simulink model "sschdlexSolarInverterSingleNetworkModel"  (R2026a)
settings: Solver=FixedStepDiscrete  StopTime=.5  MaxStep=1e-4
PreLoadFcn:
  | load('EmulatedPV_LowPowerData.mat');
  | irr = 0.15;
  | numIrr = 10;
  | ArrayPower = ArrayCurrent.*ArrayVoltage;
  | 
  | C_Boost_In = 680e-6;
  | C_Boost_In_R = 0;
  | L_Boost = 100e-6;
  | L_Boost_R = 0;
  | C_Boost_Out = 1640e-6;
  | 
  | TsFPGA = 2e-6;
  | TsControl = 2e-6;
  | TsCPU = 2e-6;
  | Tc = TsControl;
  | Ts = 2e-6;
  | 
  | IGBT_Vth = 6;
  | IGBT_Vf = 0.8;
  | IGBT_R = 0.001;
  | IGBT_Con = 1e-5;
  | 
  | IGBT_D_Vth = 0.8;
  | IGBT_D_R = 0.001;
  | IGBT_D_Con = 1e-5;
  | 
  | maxIn = 10;
  | minIn = -10;
  | maxOut = 2^15;
  | minOut = -2^15;
  | difIn = maxIn-minIn;
  | difOut = maxOut-minOut;
  | gain = difOut/difIn;
  | dc1 = (maxOut+minOut)/2;
  | dc2 = (maxIn+minIn)/2;
  | offset = dc1-gain*dc2;
  | numIrr = 10;
  | ArrayPower = ArrayCurrent.*ArrayVoltage;
InitFcn:
  | Ts = 2e-6;
  | Tc = Ts;
values from neighbouring files (symbols this model uses):
  ArrayCurrent = [3 2.90135967378 2.78442846347 2.64406556825 2.47269969012 2.25842875672 1.98100825201 1.60223040661 1.04533074246 0.222841716608 0 0 ... (1000 elements, 100x10)]    [EmulatedPV_LowPowerData.mat]
  ArrayVoltage = [0 0.151515151515 0.30303030303 0.454545454545 0.606060606061 0.757575757576 0.909090909091 1.06060606061 1.21212121212 1.36363636364 1.51515151515 1.66666666667 ... (100 elements, 100x1)]    [EmulatedPV_LowPowerData.mat]
  Irradiance = [0.05 0.1 0.15 0.2 0.25 0.3 0.35 0.4 0.45 0.5]    [EmulatedPV_LowPowerData.mat]
undefined symbols (not defined in the file or in its folder): DiscIntNeverNeededParam, ee_sli_rtmsupport, gcbh, Tdata
libraries: fl_lib x19, nesl_utility x12, eeGeneralControl x8, ee_lib x6, simulink x3, slpidlib x2
(part 1 of 2)
CloseFcn:
  | clear ArrayCurrent
  | clear ArrayVoltage
  | clear Irradiance
  | 
  | clear irr;
  | clear numIrr;
  | clear ArrayPower;
  | 
  | clear C_Boost_In;
  | clear C_Boost_In_R;
  | clear L_Boost;
  | clear L_Boost_R;
  | clear C_Boost_Out;
  | 
  | clear TsFPGA;
  | clear TsControl;
  | clear TsCPU;
  | clear Tc;
  | clear Ts;
  | 
  | clear IGBT_Vth;
  | clear IGBT_Vf;
  | clear IGBT_R ;
  | clear IGBT_Con;
  | 
  | clear IGBT_D_Vth;
  | clear IGBT_D_R;
  | clear IGBT_D_Con;
  | 
  | clear maxIn;
  | clear minIn;
  | clear maxOut;
  | clear minOut;
  | clear difIn;
  | clear difOut;
  | clear gain;
  | clear dc1;
  | clear dc2;
  | clear offset;
settings Model: DataTypeOverride=Off  Creator=The MathWorks, Inc.  LastModifiedBy=The MathWorks, Inc.
settings OptimizationCC: ConditionallyExecuteInputs=off  InheritOutputTypeSmallerThanSingle=on  EfficientMapNaN2IntZero=off
settings DebuggingCC: ArtificialAlgebraicLoopMsg=error  SingleTaskRateTransMsg=error  ParameterPrecisionLossMsg=none  PregeneratedLibrarySubsystemCodeDiagnostic=none
settings HardwareCC: ProdHWDeviceType=ASIC/FPGA->ASIC/FPGA  TargetBitPerLong=64.0  TargetBitPerPointer=64.0  TargetBitPerSizeT=64.0  TargetBitPerPtrDiffT=64.0  TargetLongLongMode=on  TargetIntDivRoundTo=Zero  TargetEndianess=LittleEndian  TargetWordSize=64.0  TargetHWDeviceType=Custom Processor->MATLAB Host Computer  ProdEqTarget=off
settings CodeAppCC: MaxIdLength=128.0
settings GRTTargetCC: CombineOutputUpdateFcns=off  GRTInterface=on
settings SimscapeCC: SimscapeNominalValues="[{\"value\":\"1\",\"unit\":\"A\"},{\"value\":\"1\",\"unit\":\"bar\"},{\"value\":\"1\",\"unit\":\"cm^2\"},{\"value\":\"1\",\"unit\":\"cm^3/s\"},{\"value\":\"1\",\"unit\":\"kJ/kg\"},{\"value\":\"1\",\"unit\":\"kW\"},{\"value\":\"1\",\"unit\":\"l\"},{\"value\":\"1\",\"unit\":\"N\"},{\"value\":\"1\",\"unit\":\"N*m\"},{\"value\":\"1\",\"unit\":\"V\"}]"  SimscapeLogType=none  SimscapeLogDataHistory=5000.0

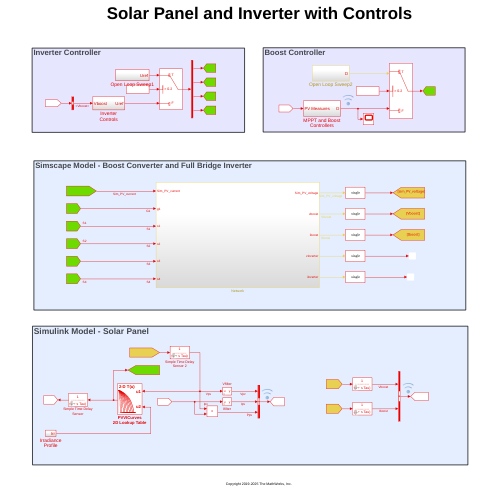
[thumbnail: Simulink's stored preview of the top-level diagram]
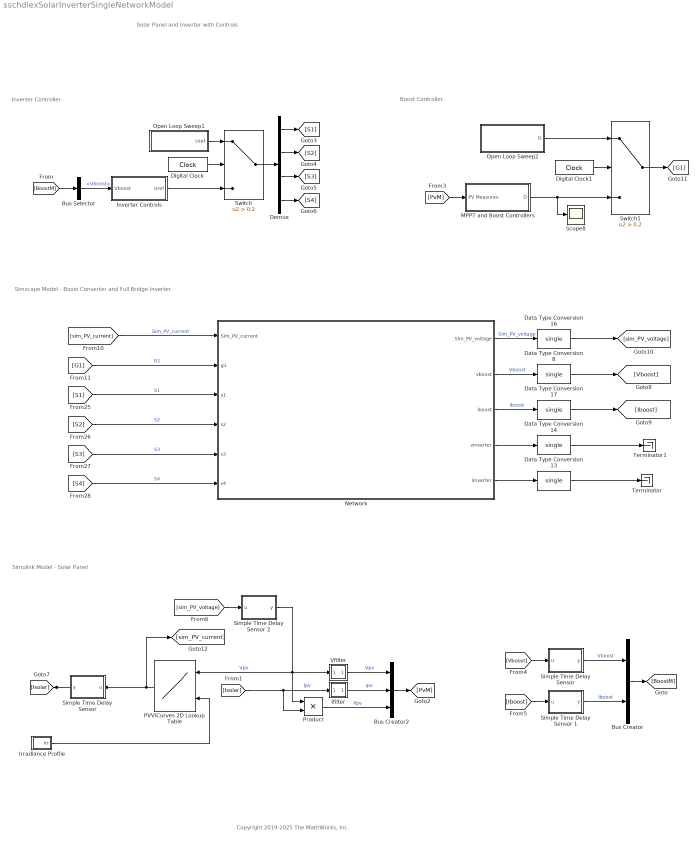
== system sschdlexSolarInverterSingleNetworkModel ==
  note: Solar Panel and Inverter with Controls
  note: Simulink Model - Solar Panel
  note: Inverter Controller
  note: Boost Controller
  note: Simscape Model - Boost Converter and Full Bridge Inverter
  note: Copyright 2019-2025 The MathWorks, Inc.
  Bus Creator : BusCreator  Inputs=2
  Bus Creator2 : BusCreator  Inputs=3
  Bus Selector : BusSelector  OutputSignals=Vboost
  Data Type Conversion{13..14,16..17} (4 alike) : DataTypeConversion  OutDataTypeStr=single  RndMeth=Nearest  SaturateOnIntegerOverflow=off
  Data Type Conversion8 : DataTypeConversion  OutDataTypeStr=single  SaturateOnIntegerOverflow=off  RndMeth=Floor
  Demux : Demux
  Digital Clock : DigitalClock  SampleTime=2e-6
  Digital Clock1 : DigitalClock  SampleTime=2e-6
  Ifilter : Subsystem  mask{Tf=0.01}
      mask prompts: Tf "Filter Time Constant"
  Inverter Controls : Subsystem
  Irradiance Profile : Subsystem
  MPPT and Boost Controllers : Subsystem
  Network : Subsystem
  Open Loop Sweep1 : Subsystem
  Open Loop Sweep2 : Subsystem
  PVVICurves 2D Lookup Table : Lookup_n-D  BreakpointsForDimension1=ArrayVoltage  BreakpointsForDimension2=Irradiance  Table=ArrayCurrent  InternalRulePriority=Speed  RndMeth=Simplest
      settings: InputPortMap=u0,u1
  Product : Product
  Scope8 : Scope
  Simple Time Delay Sensor : Subsystem  mask{Ts=Ts, Tau=0.0001}
      mask prompts: Ts "Sample Time, [s]"; Tau "Time Constant, Tau [s]"
      mask help: Simple Sensor
      mask Display: fprintf('1\n------------\n(1 + s Tau)');
  "Simple Time Delay Sensor " : Subsystem  mask{Ts=Ts, Tau=0.0001}
      mask prompts: Ts "Sample Time, [s]"; Tau "Time Constant, Tau [s]"
      mask help: Simple Sensor
      mask Display: fprintf('1\n------------\n(1 + s Tau)');
  Simple Time Delay Sensor 1 : Subsystem  mask{Ts=Ts, Tau=0.0001}
      mask prompts: Ts "Sample Time, [s]"; Tau "Time Constant, Tau [s]"
      mask help: Simple Sensor
      mask Display: fprintf('1\n------------\n(1 + s Tau)');
  Simple Time Delay Sensor 2 : Subsystem  mask{Ts=Ts, Tau=0.0001}
      mask prompts: Ts "Sample Time, [s]"; Tau "Time Constant, Tau [s]"
      mask help: Simple Sensor
      mask Display: fprintf('1\n------------\n(1 + s Tau)');
  Switch : Switch  Criteria=u2 > Threshold  Threshold=0.2  SaturateOnIntegerOverflow=off  InputSameDT=off
  Switch1 : Switch  Criteria=u2 > Threshold  Threshold=0.2  SaturateOnIntegerOverflow=off  InputSameDT=off
  Terminator : Terminator
  Terminator1 : Terminator
  Vfilter : Subsystem  mask{Tf=0.01}
      mask prompts: Tf "Filter Time Constant"
  wires:
  Bus Creator/1 -> [BoostM]
  Demux/3 -> [S3]
  Demux/2 -> [S2]
  Irradiance Profile/1(Irr) -> PVVICurves 2D Lookup Table/2
  Product/1 -> Bus Creator2/3  "Ppv"
  Vfilter/1(y) -> Bus Creator2/1  "Vpv"
  [PvM] -> MPPT and Boost Controllers/1(PV Measures)
  PVVICurves 2D Lookup Table/1 -> Simple Time Delay Sensor/1(u), [sim_PV_current]
  [sim_PV_voltage] -> Simple Time Delay Sensor 2/1(u)
  MPPT and Boost Controllers/1(D) -> Scope8/1, Switch1/3
  [Iboost] -> Simple Time Delay Sensor 1/1(u)
  Open Loop Sweep1/1(Uref) -> Switch/1
  Bus Selector/1 -> Inverter Controls/1(Vboost)  "<Vboost>"
  Digital Clock1/1 -> Switch1/2
  Ifilter/1(y) -> Bus Creator2/2  "Ipv"
  [Isolar] -> Product/2, Ifilter/1(u)  "Ipv"
  Switch/1 -> Demux/1
  Switch1/1 -> [G1]
  Simple Time Delay Sensor/1(y) -> [Isolar]
  Bus Creator2/1 -> [PvM]
  Simple Time Delay Sensor 2/1(y) -> PVVICurves 2D Lookup Table/1, Product/1, Vfilter/1(u)  "Vpv"
  Simple Time Delay Sensor 1/1(y) -> Bus Creator/2  "Iboost"
  [Vboost] -> "Simple Time Delay Sensor "/1(u)
  Demux/1 -> [S1]
  Demux/4 -> [S4]
  [BoostM] -> Bus Selector/1
  Open Loop Sweep2/1(D) -> Switch1/1
  "Simple Time Delay Sensor "/1(y) -> Bus Creator/1  "Vboost"
  Inverter Controls/1(Uref) -> Switch/3
  Digital Clock/1 -> Switch/2
  [S4] -> Network/6(s4)  "S4"
  [S2] -> Network/4(s2)  "S2"
  [S1] -> Network/3(s1)  "S1"
  Data Type Conversion8/1 -> [Vboost]
  Data Type Conversion16/1 -> [sim_PV_voltage]
  Data Type Conversion17/1 -> [Iboost]
  [sim_PV_current] -> Network/1(Sim_PV_current)  "Sim_PV_current"
  Network/1(Sim_PV_voltage) -> Data Type Conversion16/1  "Sim_PV_voltage"
  Network/3(iboost) -> Data Type Conversion17/1  "Iboost"
  Network/2(vboost) -> Data Type Conversion8/1  "Vboost"
  [G1] -> Network/2(g1)  "G1"
  Data Type Conversion13/1 -> Terminator/1
  Data Type Conversion14/1 -> Terminator1/1
  [S3] -> Network/5(s3)  "S3"
  Network/4(vinverter) -> Data Type Conversion14/1
  Network/5(iinverter) -> Data Type Conversion13/1

== system sschdlexSolarInverterSingleNetworkModel/Ifilter ==
  u : Inport
  1/T6 : Gain  Gain=1/Tf
  Discrete-Time Integrator : DiscreteIntegrator  SampleTime=Tc  ICPrevOutput=DiscIntNeverNeededParam  ICPrevScaledInput=DiscIntNeverNeededParam
  Sum1 : Sum  Inputs=|+-
  y : Outport  VectorParamsAs1DForOutWhenUnconnected=off
  wires:
  Sum1/1 -> 1/T6/1
  Discrete-Time Integrator/1 -> Sum1/2, y/1
  u/1 -> Sum1/1
  1/T6/1 -> Discrete-Time Integrator/1

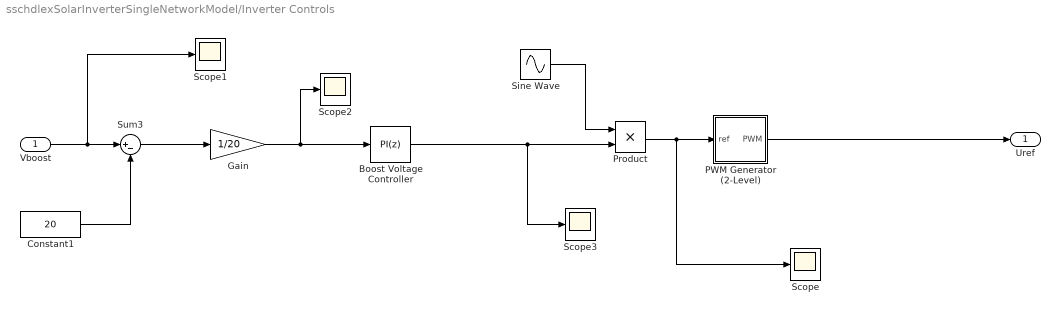
== system sschdlexSolarInverterSingleNetworkModel/Inverter Controls ==
  Vboost : Inport
  Boost Voltage Controller : slpidlib/PID Controller  Controller=PI  Form=Parallel  TimeDomain=Discrete-time  UseExternalTs=off  SampleTime=Tc  IntegratorMethod=Forward Euler  FilterMethod=Forward Euler  ControllerParametersSource=internal  P=4  I=500  UseKiTs=off  D=0  UseExternalDerivativeSource=off  N=100  UseFilter=on  TunerSelectOption=Transfer Function Based (PID Tuner App)  InitialConditionSource=internal  InitialConditionForIntegrator=1  InitialConditionForFilter=0  DifferentiatorICPrevScaledInput=0  ExternalReset=none  TrackingMode=off  Kt=1  LimitOutput=on  SatLimitsSource=internal  UpperSaturationLimit=1  LowerSaturationLimit=0  LinearizeAsGain=on  AntiWindupMode=clamping  Kb=1  LimitIntegrator=off  UpperIntegratorSaturationLimit=inf  LowerIntegratorSaturationLimit=-inf  POutMin=[]  POutMax=[]  IOutMin=[]  IOutMax=[]  DOutMin=[]  DOutMax=[]  NOutMin=[]  NOutMax=[]  SumOutMin=[]  SumOutMax=[]  SaturationOutMin=[]  SaturationOutMax=[]  PParamMin=[]  PParamMax=[]  IParamMin=[]  IParamMax=[]  DParamMin=[]  DParamMax=[]  NParamMin=[]  NParamMax=[]  KbParamMin=[]  KbParamMax=[]  KtParamMin=[]  KtParamMax=[]  KbOutMin=[]  KbOutMax=[]  KtOutMin=[]  KtOutMax=[]  IntegratorOutMin=[]  IntegratorOutMax=[]  FilterOutMin=[]  FilterOutMax=[]  SumI1OutMin=[]  SumI1OutMax=[]  SumI2OutMin=[]  SumI2OutMax=[]  SumI3OutMin=[]  SumI3OutMax=[]  SumI4OutMin=[]  SumI4OutMax=[]  SumDOutMin=[]  SumDOutMax=[]  DifferentiatorOutMin=[]  DifferentiatorOutMax=[]  FilterDiffOutCoefMin=[]  FilterDiffOutCoefMax=[]  ReciprocalOutMin=[]  ReciprocalOutMax=[]  SumDenOutMin=[]  SumDenOutMax=[]  SumNumOutMin=[]  SumNumOutMax=[]  DivideOutMin=[]  DivideOutMax=[]  UdiffTsProdOutMin=[]  UdiffTsProdOutMax=[]  NTsProdOutMin=[]  NTsProdOutMax=[]  UintegralTsProdOutMin=[]  UintegralTsProdOutMax=[]  UngainTsProdOutMin=[]  UngainTsProdOutMax=[]  ClampingZeroOutDataTypeStr=Inherit: Inherit via back propagation  ClampingZeroOutMin=[]  ClampingZeroOutMax=[]  FilterDenConstantOutDataTypeStr=Inherit: Inherit via back propagation  FilterDenConstantOutMin=[]  FilterDenConstantOutMax=[]  PCopyOutDataTypeStr=Inherit: Inherit via back propagation  PCopyOutMin=[]  PCopyOutMax=[]  NCopyOutDataTypeStr=Inherit: Inherit via back propagation  NCopyOutMin=[]  NCopyOutMax=[]  IntegratorContinuousStateAttributes=''  IntegratorStateMustResolveToSignalObject=off  IntegratorRTWStateStorageClass=Auto  FilterContinuousStateAttributes=''  FilterStateMustResolveToSignalObject=off  FilterRTWStateStorageClass=Auto  ParallelPVariant=InternalParameters  IdealPVariant=Disabled  IVariant=InternalParameters  DVariant=Disabled  IntegratorVariant=Discrete  SatVariant=Enabled  AWVariant=DiscClampingParallel  PCopyVariant=Disabled  TRVariant=Disabled  FdbkBlocksVariant=Forward  IdealPFdbkVariant=Disabled  SatFdbkVariant=Disabled  DerivativeFilterVariant=Disabled  NVariant=Disabled  NCopyVariant=Disabled_SignalSpec  FilterICVariant=Disabled  IntegratorICVariant=InternalICs  ExternalResetVariant=Disabled  TRSumVariant=Passthrough  SumFdbkVariant=Disabled  SumVariant=Sum_PI  TsampFilterVariant=InternalTs  TsampNgainVariant=Passthrough  TsampIntegralVariant=Disabled_SignalSpec  ExternalSaturationOutDataTypeStr=Inherit: Same as second input  DerivativeSourceVariant=Disabled  PreIntVariant=InternalPreInt
  Constant1 : Constant  Value=20
  Gain : Gain  Gain=1/20
  PWM Generator (2-Level) : Subsystem  mask{topology=Full-bridge, Tper=1/(2*2000), Td=1/(4*2000), Range=[-1 1], Ts=TsFPGA}
      mask prompts: topology "Converter topology"; Tper "Timer period (s)"; Td "Phase delay (s)"; Range "Output range"; Ts "Sample time"
      mask init:
      | if topology == 1
      |     PwmOutSelect = zeros(1,2);
      |     PwmOutSelect(1) = 1;
      |     PwmOutSelect(2) = 2;
      | else
      |     PwmOutSelect = zeros(1,4);
      |     PwmOutSelect(1) = 1;
      |     PwmOutSelect(2) = 2;
      |     PwmOutSelect(3) = 3;
      |     PwmOutSelect(4) = 4;
      | end
      mask TypeOptions topology: physmod:ee:library:comments:control:eePwmGeneratorMultilevel:Half0x2DBridge_PV | physmod:ee:library:comments:control:eePwmGeneratorMultilevel:Full0x2DBridge_PV
      mask TypeOptions Range: physmod:ee:library:comments:control:eeGeneralControl:x01_PV | physmod:ee:library:comments:control:eeGeneralControl:x0x2D11_PV
  Product : Product
  Scope{,1..3} (4 alike) : Scope
      Scope settings: ActiveDisplayYMinimum=-0.60405  ActiveDisplayYMaximum=0.58573  DataLoggingVariableName=ScopeData4
      Scope1 settings: ActiveDisplayYMinimum=-2.59948  ActiveDisplayYMaximum=23.39532  DataLoggingVariableName=ScopeData5
      Scope2 settings: DataLoggingVariableName=ScopeData6
      Scope3 settings: ActiveDisplayYMinimum=-0.27938  ActiveDisplayYMaximum=0.27163  DataLoggingVariableName=ScopeData7
  Sine Wave : Sin  Frequency=2*pi*60  SampleTime=Tc
  Sum3 : Sum  Inputs=|+-
  Uref : Outport  VectorParamsAs1DForOutWhenUnconnected=off
  wires:
  Constant1/1 -> Sum3/2
  Sine Wave/1 -> Product/1
  Boost Voltage Controller/1 -> Scope3/1, Product/2
  Sum3/1 -> Gain/1
  Vboost/1 -> Scope1/1, Sum3/1
  Gain/1 -> Scope2/1, Boost Voltage Controller/1
  Product/1 -> PWM Generator (2-Level)/1(ref), Scope/1
  PWM Generator (2-Level)/1(PWM) -> Uref/1

== system sschdlexSolarInverterSingleNetworkModel/Irradiance Profile ==
  note: PV Irradiance
  Irradiance : Constant  Value=0.5  OutDataTypeStr=single  SampleTime=2e-6
  Irradiance_Select : Constant  Value=0  OutDataTypeStr=single  SampleTime=2e-6
  NewIrradiance1 : Constant  Value=0.2  OutDataTypeStr=single  SampleTime=2e-6
  Pulse Generator : DiscretePulseGenerator  Amplitude=0.2  SampleTime=2e-6
  Sum : Sum  Inputs=|++
  Switch : Switch  Criteria=u2 > Threshold  SaturateOnIntegerOverflow=off  InputSameDT=off
  Irr : Outport  VectorParamsAs1DForOutWhenUnconnected=off
  wires:
  NewIrradiance1/1 -> Sum/2
  Pulse Generator/1 -> Sum/1
  Sum/1 -> Switch/3
  Irradiance/1 -> Switch/1
  Switch/1 -> Irr/1
  Irradiance_Select/1 -> Switch/2

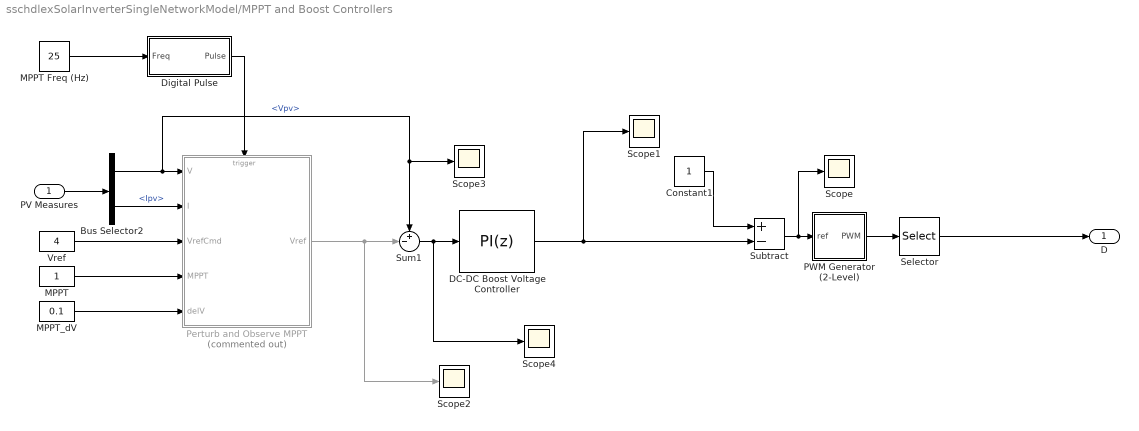
== system sschdlexSolarInverterSingleNetworkModel/MPPT and Boost Controllers ==
  PV Measures : Inport
  Bus Selector2 : BusSelector  OutputSignals=Vpv,Ipv
  Constant1 : Constant
  DC-DC Boost Voltage Controller : slpidlib/PID Controller  Controller=PI  Form=Parallel  TimeDomain=Discrete-time  UseExternalTs=off  SampleTime=Tc  IntegratorMethod=Forward Euler  FilterMethod=Forward Euler  ControllerParametersSource=internal  P=0.015  I=2.5  UseKiTs=off  D=0  UseExternalDerivativeSource=off  N=100  UseFilter=on  TunerSelectOption=Transfer Function Based (PID Tuner App)  InitialConditionSource=internal  InitialConditionForIntegrator=0  InitialConditionForFilter=0  DifferentiatorICPrevScaledInput=0  ExternalReset=none  TrackingMode=off  Kt=1  LimitOutput=off  SatLimitsSource=internal  UpperSaturationLimit=0.9  LowerSaturationLimit=0  LinearizeAsGain=on  AntiWindupMode=clamping  Kb=1  LimitIntegrator=off  UpperIntegratorSaturationLimit=inf  LowerIntegratorSaturationLimit=-inf  POutMin=[]  POutMax=[]  IOutMin=[]  IOutMax=[]  DOutMin=[]  DOutMax=[]  NOutMin=[]  NOutMax=[]  SumOutMin=[]  SumOutMax=[]  SaturationOutMin=[]  SaturationOutMax=[]  PParamMin=[]  PParamMax=[]  IParamMin=[]  IParamMax=[]  DParamMin=[]  DParamMax=[]  NParamMin=[]  NParamMax=[]  KbParamMin=[]  KbParamMax=[]  KtParamMin=[]  KtParamMax=[]  KbOutMin=[]  KbOutMax=[]  KtOutMin=[]  KtOutMax=[]  IntegratorOutMin=[]  IntegratorOutMax=[]  FilterOutMin=[]  FilterOutMax=[]  SumI1OutMin=[]  SumI1OutMax=[]  SumI2OutMin=[]  SumI2OutMax=[]  SumI3OutMin=[]  SumI3OutMax=[]  SumI4OutMin=[]  SumI4OutMax=[]  SumDOutMin=[]  SumDOutMax=[]  DifferentiatorOutMin=[]  DifferentiatorOutMax=[]  FilterDiffOutCoefMin=[]  FilterDiffOutCoefMax=[]  ReciprocalOutMin=[]  ReciprocalOutMax=[]  SumDenOutMin=[]  SumDenOutMax=[]  SumNumOutMin=[]  SumNumOutMax=[]  DivideOutMin=[]  DivideOutMax=[]  UdiffTsProdOutMin=[]  UdiffTsProdOutMax=[]  NTsProdOutMin=[]  NTsProdOutMax=[]  UintegralTsProdOutMin=[]  UintegralTsProdOutMax=[]  UngainTsProdOutMin=[]  UngainTsProdOutMax=[]  ClampingZeroOutDataTypeStr=Inherit: Inherit via back propagation  ClampingZeroOutMin=[]  ClampingZeroOutMax=[]  FilterDenConstantOutDataTypeStr=Inherit: Inherit via back propagation  FilterDenConstantOutMin=[]  FilterDenConstantOutMax=[]  PCopyOutDataTypeStr=Inherit: Inherit via back propagation  PCopyOutMin=[]  PCopyOutMax=[]  NCopyOutDataTypeStr=Inherit: Inherit via back propagation  NCopyOutMin=[]  NCopyOutMax=[]  IntegratorContinuousStateAttributes=''  IntegratorStateMustResolveToSignalObject=off  IntegratorRTWStateStorageClass=Auto  FilterContinuousStateAttributes=''  FilterStateMustResolveToSignalObject=off  FilterRTWStateStorageClass=Auto  ParallelPVariant=InternalParameters  IdealPVariant=Disabled  IVariant=InternalParameters  DVariant=Disabled  IntegratorVariant=Discrete  SatVariant=Disabled  AWVariant=Passthrough  PCopyVariant=Disabled  TRVariant=Disabled  FdbkBlocksVariant=Forward  IdealPFdbkVariant=Disabled  SatFdbkVariant=Disabled  DerivativeFilterVariant=Disabled  NVariant=Disabled  NCopyVariant=Disabled_SignalSpec  FilterICVariant=Disabled  IntegratorICVariant=InternalICs  ExternalResetVariant=Disabled  TRSumVariant=Passthrough  SumFdbkVariant=Disabled  SumVariant=Sum_PI  TsampFilterVariant=InternalTs  TsampNgainVariant=Passthrough  TsampIntegralVariant=Disabled_SignalSpec  ExternalSaturationOutDataTypeStr=Inherit: Same as second input  DerivativeSourceVariant=Disabled  PreIntVariant=InternalPreInt
  Digital Pulse : Subsystem  mask{Ts=Tc, Duty=0.5}
      mask prompts: Ts "Sample Rate [s]"; Duty "Duty Cycle [0-1]"
  MPPT : Constant
  MPPT Freq (Hz) : Constant  Value=25
  MPPT_dV : Constant  Value=0.1
  PWM Generator (2-Level) : Subsystem  mask{topology=Full-bridge, Tper=1/(2*2000), Td=1/(4*2000), Range=[0 1], Ts=TsFPGA}
      mask prompts: topology "Converter topology"; Tper "Timer period (s)"; Td "Phase delay (s)"; Range "Output range"; Ts "Sample time"
      mask init: same as sschdlexSolarInverterSingleNetworkModel/Inverter Controls/PWM Generator (2-Level)
      mask TypeOptions topology: physmod:ee:library:comments:control:eePwmGeneratorMultilevel:Half0x2DBridge_PV | physmod:ee:library:comments:control:eePwmGeneratorMultilevel:Full0x2DBridge_PV
      mask TypeOptions Range: physmod:ee:library:comments:control:eeGeneralControl:x01_PV | physmod:ee:library:comments:control:eeGeneralControl:x0x2D11_PV
  Perturb and Observe MPPT : Subsystem  Commented=on  TreatAsAtomicUnit=on  SystemSampleTime=Tdata
  Scope{,1..4} (5 alike) : Scope
      Scope settings: ActiveDisplayYMinimum=0.51551  ActiveDisplayYMaximum=1.23833
      Scope1 settings: ActiveDisplayYMinimum=-0.23833  ActiveDisplayYMaximum=0.48449  DataLoggingVariableName=ScopeData2
      Scope2 settings: ActiveDisplayYMinimum=4.975  ActiveDisplayYMaximum=5.225
      Scope3 settings: ActiveDisplayYMinimum=-1.20462  ActiveDisplayYMaximum=10.84161  DataLoggingVariableName=ScopeData2
      Scope4 settings: ActiveDisplayYMinimum=-6.20462  ActiveDisplayYMaximum=5.84161  DataLoggingVariableName=ScopeData3
  Selector : Selector  InputPortWidth=4  IndexOptions=Index vector (dialog)  Indices=2  OutputSizes=1
  Subtract : Sum  Inputs=+-
  Sum1 : Sum  Inputs=+-|
  Vref : Constant  Value=4
  D : Outport  VectorParamsAs1DForOutWhenUnconnected=off
  wires:
  PV Measures/1 -> Bus Selector2/1
  Digital Pulse/1(Pulse) -> Perturb and Observe MPPT/Trigger
  MPPT Freq (Hz)/1 -> Digital Pulse/1(Freq)
  MPPT_dV/1 -> Perturb and Observe MPPT/5(delV)
  Vref/1 -> Perturb and Observe MPPT/3(VrefCmd)
  Sum1/1 -> Scope4/1, DC-DC Boost Voltage Controller/1
  MPPT/1 -> Perturb and Observe MPPT/4(MPPT)
  Bus Selector2/1 -> Perturb and Observe MPPT/1(V), Scope3/1, Sum1/1  "<Vpv>"
  Perturb and Observe MPPT/1(Vref) -> Scope2/1, Sum1/2
  Bus Selector2/2 -> Perturb and Observe MPPT/2(I)  "<Ipv>"
  Selector/1 -> D/1
  PWM Generator (2-Level)/1(PWM) -> Selector/1
  Constant1/1 -> Subtract/1
  DC-DC Boost Voltage Controller/1 -> Scope1/1, Subtract/2
  Subtract/1 -> PWM Generator (2-Level)/1(ref), Scope/1

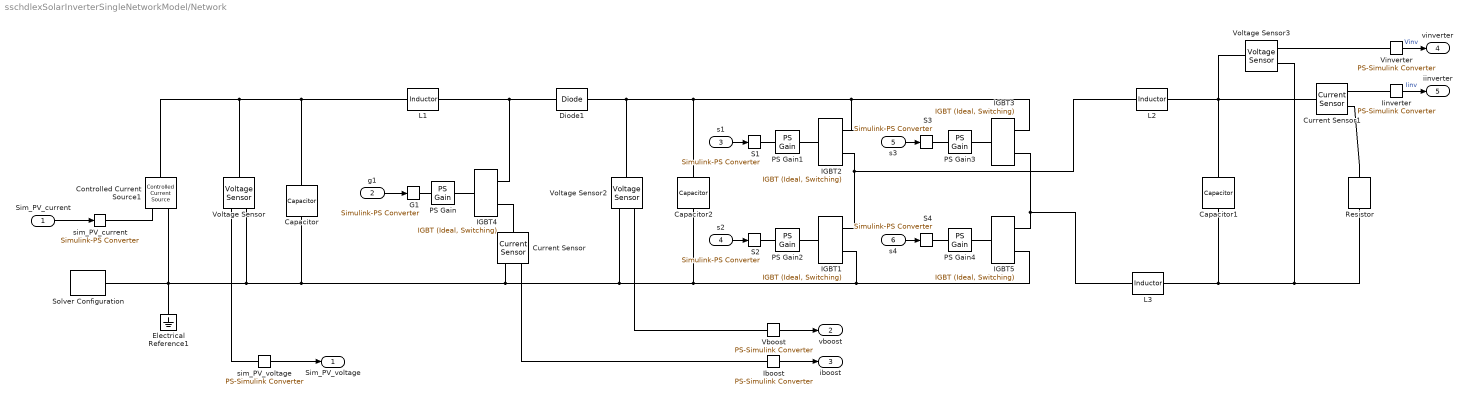
== system sschdlexSolarInverterSingleNetworkModel/Network ==
  Sim_PV_current : Inport
  g1 : Inport  Port=2
  s1 : Inport  Port=3
  s2 : Inport  Port=4
  s3 : Inport  Port=5
  s4 : Inport  Port=6
  Capacitor : fl_lib/Electrical/Electrical Elements/Capacitor  c=C_Boost_In F  r=C_Boost_In_R Ohm  g=0 1/Ohm  i_specify=off  i_priority=None  i=0 A  i_nominal_specify=off  i_nominal_value=1  i_nominal_unit=A  v_specify=off  v_priority=None  v=0 V  v_nominal_specify=off  v_nominal_value=1  v_nominal_unit=V  vc_specify=off  vc_priority=High  vc=0 V  vc_nominal_specify=off  vc_nominal_value=1  vc_nominal_unit=V
  Capacitor1 : fl_lib/Electrical/Electrical Elements/Capacitor  c=3e-6 F  r=0 Ohm  g=0 1/Ohm  i_specify=off  i_priority=None  i=0 A  i_nominal_specify=off  i_nominal_value=1  i_nominal_unit=A  v_specify=off  v_priority=None  v=0 V  v_nominal_specify=off  v_nominal_value=1  v_nominal_unit=V  vc_specify=off  vc_priority=High  vc=0 V  vc_nominal_specify=off  vc_nominal_value=1  vc_nominal_unit=V
  Capacitor2 : fl_lib/Electrical/Electrical Elements/Capacitor  c=2*1640e-6 F  r=0.0005 Ohm  g=0 1/Ohm  i_specify=off  i_priority=None  i=0 A  i_nominal_specify=off  i_nominal_value=1  i_nominal_unit=A  v_specify=off  v_priority=None  v=0 V  v_nominal_specify=off  v_nominal_value=1  v_nominal_unit=V  vc_specify=off  vc_priority=High  vc=0 V  vc_nominal_specify=off  vc_nominal_value=1  vc_nominal_unit=V
  Controlled Current Source1 : fl_lib/Electrical/Electrical Sources/Controlled Current Source
  Current Sensor : fl_lib/Electrical/Electrical Sensors/Current Sensor
  Current Sensor1 : fl_lib/Electrical/Electrical Sensors/Current Sensor
  Diode1 : ee_lib/Semiconductors & Converters/Diode  ModelType=ee.enum.diode.modelType.pwl  TableType=ee.enum.diode.tableType.IfMat  IfMat=[.07, .12, .19, 1.75, 4.24, 7.32, 11.2; .16, .3, .72, 2.14, 5.02, 8.35, 13.12] A  VfMat=[.9, 1.15, 1.25, 1.5, 1.75, 2.17, 2.6, 2.85; .58, .68, .75, 1.1, 1.38, 1.77, 2.27, 2.7] V  TjVec=[25, 125] degC  VfVec=[.5, .7, .9, 1.3, 1.7, 2.1, 2.5] V  IfVec=[.1, .2, .5, 1, 2, 4, 7, 10] A  IrMat=[1e-06, 2e-06, 5e-06, 1e-05, 2.5e-05, 5e-05, .0001; 2e-06, 5e-06, 1e-05, 4e-05, 8e-05, .0002, .0005] A  VrMat=[10, 100, 200, 250, 300, 325, 350; 10, 70, 160, 220, 270, 300, 320] V  VrVec=[10, 20, 40, 50, 70, 80, 100] V  IrVec=[1e-06, 2e-06, 5e-06, 1e-05, 2e-05, 5e-05, .0001] A  Vf=0.8 V  Ron=0.001 Ohm  Goff=1e-8 S  prmExp=ee.enum.diode.expParam.useTwo  I12=[.0137, .545] A  V12=[.6, .7] V  RS=0 Ohm  Tmeas=25 degC  IS=1e-12 A  ec=1  I1=0.0137 A  V1=0.6 V  N_series=1  N_parallel=1  ZenerEnable=false  Rz=0.3 Ohm  BV=inf V  C_param=ee.enum.diode.capParam.fixed  CJ=0 pF  CJ0=5 pF  Vvec=[.1, 10, 100] V  Cvec=[3.5, 1, .4] pF  VJ=1 V  Mgrad=0.5  FC=0.5  Q_param=ee.enum.diode.recoveryParam.off  iRM=-7.15 A  iF=4 A  didt=-750 A/us  trr_factor=3  trr=115 ns  Qrr=150 nA*s  Vr=-600 V  Ls=150 nH  Erec=0.03 J  TT=50 ns  tau=100 ns  T_param=ee.enum.diode.temperatureParam.off  Tdevice=25 degC  I1_T2=0.245 A  V1_T2=0.5 V  IS_T2=1.25e-7 A  Tmeas2=125 degC  XTI_param=ee.enum.diode.xtiParam.pn  XTI=3  EG_param=ee.enum.diode.egapParam.material_si  EG=1.11 eV  dBVdT=0 V/K  enable_fault_input=simscape.enum.onoff.off  i_specify=off  i_priority=None  i=0 A  i_nominal_specify=off  i_nominal_value=1  i_nominal_unit=A  v_specify=off  v_priority=None  v=0 V  v_nominal_specify=off  v_nominal_value=1  v_nominal_unit=V  v_capacitor_specify=off  v_capacitor_priority=None  v_capacitor=0 V  v_capacitor_nominal_specify=off  v_capacitor_nominal_value=1  v_capacitor_nominal_unit=V  Qj_specify=off  Qj_priority=High  Qj=0 C  Qj_nominal_specify=off  Qj_nominal_value=1  Qj_nominal_unit=C  i_diode_specify=off  i_diode_priority=None  i_diode=0 A  i_diode_nominal_specify=off  i_diode_nominal_value=1  i_diode_nominal_unit=A  v_diode_specify=off  v_diode_priority=None  v_diode=0 V  v_diode_nominal_specify=off  v_diode_nominal_value=1  v_diode_nominal_unit=V  i_capacitor_specify=off  i_capacitor_priority=None  i_capacitor=0 A  i_capacitor_nominal_specify=off  i_capacitor_nominal_value=1  i_capacitor_nominal_unit=A  fidelity_level=ee.enum.diode.fidelity.includeChargeDyn  rec_loss_model=ee.enum.diode.reverseRecoveryModel.fixed  ErecVal=0 J  scaleWithIandV=true  ErecMat=zeros(2, 3) J  ErecMat3D=zeros(2, 3, 2) J  TjrecVec=[298.15, 398.15] K  IfrecVec=[.1, 1, 10] A  IrecVal=10 A  VrecVal=10 V  VrecVec=[0, 100] V  tFilter=1 / 1000 / 100 s  thermal_network_parameterization=ee.enum.thermalNetworkTopology.junctionCase  Rth=[0, 10] K/W  Rth_Cauer=[1, 3, 10] K/W  Rth_Foster=[4, 6] K/W  thermal_mass_parameterization=ee.enum.thermalNetwork.timeconstant  thermal_mass=[0, 1] J/K  thermal_mass_Cauer=[.1, .3, 1] J/K  thermal_mass_Foster=[1.5, 3] J/K  thermal_time_constant=[0, 10] s  thermal_time_constant_Cauer=[1, 3, 10] s  thermal_time_constant_Foster=[6, 18] s  thermal_mass_initial_temperatures=[25, 25] degC  thermal_mass_initial_temperatures_Cauer=[25, 25, 25] degC  junction_thermal_mass=0.01 J/K  Tvec_initial_Foster=[25, 25, 25, 25] degC  no_thermal_network=0  junction_temperature_specify=off  junction_temperature_priority=None  junction_temperature=25 degC  junction_temperature_nominal_specify=off  junction_temperature_nominal_value=1  junction_temperature_nominal_unit=degC
  Electrical Reference1 : fl_lib/Electrical/Electrical Elements/Electrical Reference
  G1 : nesl_utility/Simulink-PS Converter  PhysicalDomain=network_engine_domain  SubClassName=ps_input  LeftPortType=input  RightPortType=output  PseudoPeriodic=off  Frequencies=[]  NoiseDistribution=none  NoiseParameters=[]  Unit=1  AffineConversion=off  FilteringAndDerivatives=provide  SimscapeFilterOrder=1  InputFilterTimeConstant=0.001  UdotUserProvided=0
  IGBT{1..5} (5 alike) : ee_lib/Semiconductors & Converters/IGBT (Ideal, Switching)  port_option=ee.enum.controlport.ps  Vf=IGBT_Vf V  Ron=IGBT_R Ohm  Goff=IGBT_Con 1/Ohm  Vth=IGBT_Vth V  diode_param=2  diode_Vf=IGBT_D_Vth V  diode_Ron=IGBT_D_R Ohm  diode_Goff=IGBT_D_Con 1/Ohm  diode_C=5e-8 F  diode_iRM=-235 A  diode_iF=300 A  diode_idot=-50 A/us  diode_trr_param=1  diode_trr_factor=3  diode_trr=15 us  diode_Qrr=1.5e+3 s*uA  ice_specify=off  ice_priority=None  ice=0 A  ice_nominal_specify=off  ice_nominal_value=1  ice_nominal_unit=A  vce_specify=off  vce_priority=None  vce=0 V  vce_nominal_specify=off  vce_nominal_value=1  vce_nominal_unit=V  vge_specify=off  vge_priority=None  vge=0 V  vge_nominal_specify=off  vge_nominal_value=1  vge_nominal_unit=V  thermal_loss_option=ee.enum.converters.thermalLossOption.constantvalues  Von_data=[0, .1, .6, .8, 1, 1.3, 1.6, 2, 2.4; 0, .1, .7, 1, 1.2, 1.5, 1.9, 2.4, 2.8] V  Tj=[298.15, 398.15] K  Iout_data=[0, .1, 1, 5, 10, 20, 40, 70, 100] A  tabulateWithVce=false  Eon_data=[0, .0024, .024, .12, .2, .48, 1.04, 2.16, 3.24; 0, .003, .03, .15, .25, .6, 1.3, 2.7, 4.05] * 1e-3 J  Eoff_data=[0, .0007, .0066, .033, .066, .17, .33, .83, 1.5; 0, .001, .01, .05, .1, .25, .5, 1.2, 2.2] * 1e-3 J  Eon_data_3D=[zeros(2, 9, 3)] J  Eoff_data_3D=[zeros(2, 9, 3)] J  Tj_loss=[298.15, 398.15] K  Iout_data_loss=[0, .1, 1, 5, 10, 20, 40, 70, 100] A  Vce_loss=[0, 150, 300] V  Eon_scalar=22.86e-3 J  Eoff_scalar=17.14e-3 J  Voff=300 V  Iout_scalar=600 A  useCurrentFromPreviousCycle=false  useVoltageFromPreviousCycle=false  diodeModelType=ee.enum.converters.diodeModelType.pwl  diodeTableType=ee.enum.diode.tableType.IfMat  diode_ReverseIVType=ee.enum.diode.diodeReverseIV.constant  diode_IfMat=[.07, .12, .19, 1.75, 4.24, 7.32, 11.2; .16, .3, .72, 2.14, 4.02, 6.35, 9.12] A  diode_VfMat=[.9, 1.15, 1.25, 1.5, 1.75, 2.17, 2.6, 2.85; .58, .68, .75, 1.1, 1.38, 1.77, 2.27, 2.7] V  diode_TjVec=[25, 125] degC  diode_VfVec=[.5, .7, .9, 1.3, 1.7, 2.1, 2.5] V  diode_IfVec=[.1, .2, .5, 1, 2, 4, 7, 10] A  diode_IrMat=[1e-06, 2e-06, 5e-06, 1e-05, 2.5e-05, 5e-05, .0001; 2e-06, 5e-06, 1e-05, 4e-05, 8e-05, .0002, .0005] A  diode_VrMat=[10, 100, 200, 250, 300, 325, 350; 10, 70, 160, 220, 270, 300, 320] V  diode_VrVec=[10, 20, 40, 50, 70, 80, 100] V  diode_IrVec=[1e-06, 2e-06, 5e-06, 1e-05, 2e-05, 5e-05, .0001] A  diode_Vr=-600 V  diode_Ls=150 nH  diode_Erec=0.03 J  diode_rec_loss_model=ee.enum.diode.reverseRecoveryModel.fixed  diode_ErecVal=0 J  diode_scaleWithIandV=true  diode_ErecMat=zeros(2, 3) J  diodeErecMat3D=zeros(2, 3, 2) J  diode_TjrecVec=[298.15, 398.15] K  diode_IfrecVec=[.1, 1, 10] A  diodeVrecVec=[0, 100] V  diode_IrecVal=10 A  diode_VrecVal=10 V  diode_tFilter=1 / 1000 / 100 s  separateThermalPortForDiode=false  thermal_network_parameterization=ee.enum.thermalNetworkTopology.external  Rth=[.08, .5] K/W  Rth_Cauer=[.08, .1, .5] K/W  Rth_Foster=[.08, .14, .22, .16] K/W  thermal_mass_parameterization=ee.enum.thermalNetwork.timeconstant  thermal_mass=[.01, .5] J/K  thermal_mass_Cauer=[.01, .1, .5] J/K  thermal_mass_Foster=[.001, .005, .05, .5] J/K  thermal_time_constant=[.001, .2] s  thermal_time_constant_Cauer=[.001, .1, .2] s  thermal_time_constant_Foster=[7e-05, .0007, .01, .08] s  thermal_mass_initial_temperatures=[25, 25] degC  thermal_mass_initial_temperatures_Cauer=[25, 25, 25] degC  junction_thermal_mass=0.01 J/K  Tvec_initial_Foster=[25, 25, 25, 25] degC  RthDiode=[.03, .2] K/W  RthCauerDiode=[.03, .1, .2] K/W  RthFosterDiode=[.03, .2] K/W  thermalMassDiode=[3, 25] J/K  thermalMassCauerDiode=[3, 10, 25] J/K  thermalMassFosterDiode=[33, 50] J/K  thermalTauDiode=[.1, 5] s  thermalTauCauerDiode=[.1, 1, 5] s  thermalTauFosterDiode=[1, 10] s  thermalMassInitTempDiode=[25, 25] degC  thermalMassInitTempCauerDiode=[25, 25, 25] degC  junctionthermalMassDiode=0.1 J/K  TVecInitialFosterDiode=[25, 25, 25, 25] degC  no_thermal_network=0  IGBT_junction_temperature_specify=off  IGBT_junction_temperature_priority=None  IGBT_junction_temperature=25 degC  IGBT_junction_temperature_nominal_specify=off  IGBT_junction_temperature_nominal_value=1  IGBT_junction_temperature_nominal_unit=degC  diode_junction_temperature_specify=off  diode_junction_temperature_priority=None  diode_junction_temperature=25 degC  diode_junction_temperature_nominal_specify=off  diode_junction_temperature_nominal_value=1  diode_junction_temperature_nominal_unit=degC  Qj_specify=off  Qj_priority=None  Qj=0 W  Qj_nominal_specify=off  Qj_nominal_value=1  Qj_nominal_unit=W  accumulatedSwitchingLosses_specify=off  accumulatedSwitchingLosses_priority=None  accumulatedSwitchingLosses=0 J
  Iboost : nesl_utility/PS-Simulink Converter  PhysicalDomain=network_engine_domain  SubClassName=ps_output  LeftPortType=input  RightPortType=output  PseudoPeriodic=off  Frequencies=[]  VectorFormat=1-D array  Unit=1  AffineConversion=off
  Iinverter : nesl_utility/PS-Simulink Converter  PhysicalDomain=network_engine_domain  SubClassName=ps_output  LeftPortType=input  RightPortType=output  PseudoPeriodic=off  Frequencies=[]  VectorFormat=1-D array  Unit=1  AffineConversion=off
  L1 : fl_lib/Electrical/Electrical Elements/Inductor  l=L_Boost H  r=L_Boost_R Ohm  g=1e-9 1/Ohm  i_specify=off  i_priority=None  i=0 A  i_nominal_specify=off  i_nominal_value=1  i_nominal_unit=A  v_specify=off  v_priority=None  v=0 V  v_nominal_specify=off  v_nominal_value=1  v_nominal_unit=V  i_L_specify=off  i_L_priority=High  i_L=0 A  i_L_nominal_specify=off  i_L_nominal_value=1  i_L_nominal_unit=A
      settings: AttributesFormatString=|
      | %<l> H
      | %<r> Ohm
  L2 : fl_lib/Electrical/Electrical Elements/Inductor  l=100e-6 H  r=0.001 Ohm  g=1e-9 1/Ohm  i_specify=off  i_priority=None  i=0 A  i_nominal_specify=off  i_nominal_value=1  i_nominal_unit=A  v_specify=off  v_priority=None  v=0 V  v_nominal_specify=off  v_nominal_value=1  v_nominal_unit=V  i_L_specify=off  i_L_priority=High  i_L=0 A  i_L_nominal_specify=off  i_L_nominal_value=1  i_L_nominal_unit=A
      settings: AttributesFormatString=|
      | %<l> H
      | %<r> Ohm
  L3 : fl_lib/Electrical/Electrical Elements/Inductor  l=100e-6 H  r=0.001 Ohm  g=1e-9 1/Ohm  i_specify=off  i_priority=None  i=0 A  i_nominal_specify=off  i_nominal_value=1  i_nominal_unit=A  v_specify=off  v_priority=None  v=0 V  v_nominal_specify=off  v_nominal_value=1  v_nominal_unit=V  i_L_specify=off  i_L_priority=High  i_L=0 A  i_L_nominal_specify=off  i_L_nominal_value=1  i_L_nominal_unit=A
      settings: AttributesFormatString=|
      | %<l> H
      | %<r> Ohm
  PS Gain{,1..4} (5 alike) : fl_lib/Physical Signals/Functions/PS Gain  gain=1.5*IGBT_Vth
  Resistor : fl_lib/Electrical/Electrical Elements/Resistor  R=11.5 Ohm  i_specify=off  i_priority=None  i=0 A  i_nominal_specify=off  i_nominal_value=1  i_nominal_unit=A  v_specify=off  v_priority=None  v=0 V  v_nominal_specify=off  v_nominal_value=1  v_nominal_unit=V
  S{1..4} (4 alike) : nesl_utility/Simulink-PS Converter  PhysicalDomain=network_engine_domain  SubClassName=ps_input  LeftPortType=input  RightPortType=output  PseudoPeriodic=off  Frequencies=[]  NoiseDistribution=none  NoiseParameters=[]  Unit=1  AffineConversion=off  FilteringAndDerivatives=provide  SimscapeFilterOrder=1  InputFilterTimeConstant=0.001  UdotUserProvided=0
  Solver Configuration : nesl_utility/Solver Configuration  PhysicalDomain=network_engine_domain  SubClassName=solver  LeftPortType=input  RightPortType=generic  Tones=[]  Harmonics=[]  SimulateNoise=off  Profile=off  UseLocalSampling=off  EnableSwitchedLinearOptims=on  FrequencyDomain=off  UseCCode=off  RelTol=0.001  AbsTol=1e-06  MinStep=1e-09  ToWorkspace=off  RevertToSquareIcSolve=off  NumHomotopyIterations=100  PhasorMode=off  PhasorModeNumHarmonics=1  ConsistencySolver=NEWTON_FTOL  CanonicalOrdering=UNORDERED  OptimizeIntermediates=UNOPTIMIZED  IndexReductionMethod=DerivativeReplacement  DoDC=off  ResidualTolerance=1e-09  ConsistencyTolSource=GLOBAL  ConsistencyAbsTol=0.001  ConsistencyRelTol=0.001  ConsistencyTolFactor=0.001  UseLocalSolver=on  LocalSolverChoice=NE_BACKWARD_EULER_ADVANCER  ResolveIndetEquations=on  FunctionEvalNumThread=1  LocalSolverSampleTime=2e-6  DoFixedCost=off  MaxNonlinIter=3  MaxModeIter=2  ComputeImpulses=off  ImpulseIterations=2  LinearAlgebra=auto  LinearAlgebraNumThread=0  EquationFormulation=NE_TIME_EF  DelaysMemoryBudget=1024  AutomaticFiltering=on  FilteringTimeConstant=0.001  PartitionStorageMethod=AS_NEEDED  PartitionMemoryBudget=1024  PartitionMethod=FAST  MultibodyUseLocalSolver=off  MultibodyLocalSolverChoice=ODE1  MultibodyLocalSolverSampleTime=0.001
  Vboost : nesl_utility/PS-Simulink Converter  PhysicalDomain=network_engine_domain  SubClassName=ps_output  LeftPortType=input  RightPortType=output  PseudoPeriodic=off  Frequencies=[]  VectorFormat=1-D array  Unit=1  AffineConversion=off
  Vinverter : nesl_utility/PS-Simulink Converter  PhysicalDomain=network_engine_domain  SubClassName=ps_output  LeftPortType=input  RightPortType=output  PseudoPeriodic=off  Frequencies=[]  VectorFormat=1-D array  Unit=1  AffineConversion=off
  Voltage Sensor : fl_lib/Electrical/Electrical Sensors/Voltage Sensor
  Voltage Sensor2 : fl_lib/Electrical/Electrical Sensors/Voltage Sensor
  Voltage Sensor3 : fl_lib/Electrical/Electrical Sensors/Voltage Sensor
  sim_PV_current : nesl_utility/Simulink-PS Converter  PhysicalDomain=network_engine_domain  SubClassName=ps_input  LeftPortType=input  RightPortType=output  PseudoPeriodic=off  Frequencies=[]  NoiseDistribution=none  NoiseParameters=[]  Unit=1  AffineConversion=off  FilteringAndDerivatives=provide  SimscapeFilterOrder=1  InputFilterTimeConstant=0.001  UdotUserProvided=0
  sim_PV_voltage : nesl_utility/PS-Simulink Converter  PhysicalDomain=network_engine_domain  SubClassName=ps_output  LeftPortType=input  RightPortType=output  PseudoPeriodic=off  Frequencies=[]  VectorFormat=1-D array  Unit=1  AffineConversion=off
  Sim_PV_voltage : Outport
  vboost : Outport  Port=2
  iboost : Outport  Port=3
  vinverter : Outport  Port=4
  iinverter : Outport  Port=5
  wires:
  s1/1 -> S1/1
  Iinverter/1 -> iinverter/1  "Iinv"
  Sim_PV_current/1 -> sim_PV_current/1
  g1/1 -> G1/1
  s4/1 -> S4/1
  s3/1 -> S3/1
  Vboost/1 -> vboost/1
  Iboost/1 -> iboost/1
  Vinverter/1 -> vinverter/1  "Vinv"
  s2/1 -> S2/1
  sim_PV_voltage/1 -> Sim_PV_voltage/1
  connections:
  Capacitor/RConn1 -- Controlled Current Source1/RConn2 -- Electrical Reference1/LConn1 -- Solver Configuration/RConn1 -- Voltage Sensor/RConn2 -- IGBT5/RConn2 -- IGBT1/RConn2 -- Capacitor2/RConn1 -- Voltage Sensor2/RConn2 -- Current Sensor/RConn2
  L1/RConn1 -- Diode1/LConn1 -- IGBT4/RConn1
  Voltage Sensor3/RConn2 -- Resistor/RConn1 -- Capacitor1/RConn1 -- L3/RConn1
  Voltage Sensor2/LConn1 -- Diode1/RConn1 -- IGBT3/RConn1 -- IGBT2/RConn1 -- Capacitor2/LConn1
  IGBT3/RConn2 -- L3/LConn1 -- IGBT5/RConn1
  L1/LConn1 -- Controlled Current Source1/LConn1 -- Voltage Sensor/LConn1 -- Capacitor/LConn1
  IGBT1/RConn1 -- L2/LConn1 -- IGBT2/RConn2
  Capacitor1/LConn1 -- Current Sensor1/LConn1 -- L2/RConn1 -- Voltage Sensor3/LConn1
  PS Gain4/LConn1 -- S4/RConn1
  PS Gain3/LConn1 -- S3/RConn1
  Current Sensor/RConn1 -- Iboost/LConn1
  Resistor/LConn1 -- Current Sensor1/RConn2
  PS Gain1/LConn1 -- S1/RConn1
  PS Gain2/LConn1 -- S2/RConn1
  Voltage Sensor2/RConn1 -- Vboost/LConn1
  IGBT1/LConn1 -- PS Gain2/RConn1
  IGBT3/LConn1 -- PS Gain3/RConn1
  PS Gain/RConn1 -- IGBT4/LConn1
  IGBT5/LConn1 -- PS Gain4/RConn1
  Iinverter/LConn1 -- Current Sensor1/RConn1
  Voltage Sensor3/RConn1 -- Vinverter/LConn1
  Controlled Current Source1/RConn1 -- sim_PV_current/RConn1
  sim_PV_voltage/LConn1 -- Voltage Sensor/RConn1
  G1/RConn1 -- PS Gain/LConn1
  IGBT2/LConn1 -- PS Gain1/RConn1
  IGBT4/RConn2 -- Current Sensor/LConn1

== system sschdlexSolarInverterSingleNetworkModel/Open Loop Sweep1 ==
  Constant : Constant
  PWM Generator (2-Level) : Subsystem  mask{topology=Full-bridge, Tper=1/(2*2000), Td=1/(4*2000), Range=[-1 1], Ts=TsFPGA}
      mask prompts: topology "Converter topology"; Tper "Timer period (s)"; Td "Phase delay (s)"; Range "Output range"; Ts "Sample time"
      mask init: same as sschdlexSolarInverterSingleNetworkModel/Inverter Controls/PWM Generator (2-Level)
      mask TypeOptions topology: physmod:ee:library:comments:control:eePwmGeneratorMultilevel:Half0x2DBridge_PV | physmod:ee:library:comments:control:eePwmGeneratorMultilevel:Full0x2DBridge_PV
      mask TypeOptions Range: physmod:ee:library:comments:control:eeGeneralControl:x01_PV | physmod:ee:library:comments:control:eeGeneralControl:x0x2D11_PV
  Product : Product
  Sine Wave : Sin  Amplitude=0.9  Frequency=2*pi*60*2  SampleTime=Tc
  Uref : Outport  VectorParamsAs1DForOutWhenUnconnected=off
  wires:
  Product/1 -> PWM Generator (2-Level)/1(ref)
  Constant/1 -> Product/2
  Sine Wave/1 -> Product/1
  PWM Generator (2-Level)/1(PWM) -> Uref/1

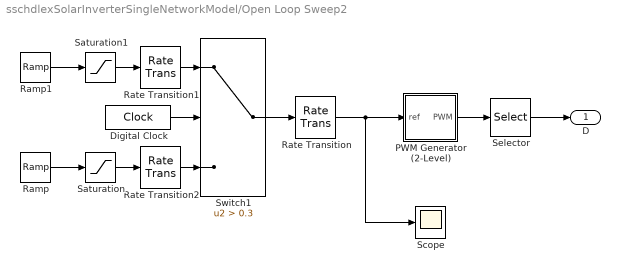
== system sschdlexSolarInverterSingleNetworkModel/Open Loop Sweep2 ==
  Digital Clock : DigitalClock  SampleTime=2e-6
  PWM Generator (2-Level) : Subsystem  mask{topology=Full-bridge, Tper=1/(2*2000), Td=1/(4*2000), Range=[0 1], Ts=TsFPGA}
      mask prompts: topology "Converter topology"; Tper "Timer period (s)"; Td "Phase delay (s)"; Range "Output range"; Ts "Sample time"
      mask init: same as sschdlexSolarInverterSingleNetworkModel/Inverter Controls/PWM Generator (2-Level)
      mask TypeOptions topology: physmod:ee:library:comments:control:eePwmGeneratorMultilevel:Half0x2DBridge_PV | physmod:ee:library:comments:control:eePwmGeneratorMultilevel:Full0x2DBridge_PV
      mask TypeOptions Range: physmod:ee:library:comments:control:eeGeneralControl:x01_PV | physmod:ee:library:comments:control:eeGeneralControl:x0x2D11_PV
  Ramp : simulink/Sources/Ramp  slope=8  start=0.2  InitialOutput=0.1
  Ramp1 : simulink/Sources/Ramp  slope=8  start=0.3  InitialOutput=0.1
  Rate Transition : RateTransition  OutPortSampleTime=2e-6
  Rate Transition1 : RateTransition  OutPortSampleTime=2e-6
  Rate Transition2 : RateTransition  OutPortSampleTime=2e-6
  Saturation : Saturate  UpperLimit=1  LowerLimit=0
  Saturation1 : Saturate  UpperLimit=1  LowerLimit=0
  Scope : Scope
      settings: ActiveDisplayYMinimum=0  ActiveDisplayYMaximum=1
  Selector : Selector  InputPortWidth=4  IndexOptions=Index vector (dialog)  Indices=2  OutputSizes=1
  Switch1 : Switch  Criteria=u2 > Threshold  Threshold=0.3  SaturateOnIntegerOverflow=off  InputSameDT=off
  D : Outport  VectorParamsAs1DForOutWhenUnconnected=off
  wires:
  Ramp/1 -> Saturation/1
  Selector/1 -> D/1
  PWM Generator (2-Level)/1(PWM) -> Selector/1
  Switch1/1 -> Rate Transition/1
  Digital Clock/1 -> Switch1/2
  Ramp1/1 -> Saturation1/1
  Saturation1/1 -> Rate Transition1/1
  Saturation/1 -> Rate Transition2/1
  Rate Transition/1 -> PWM Generator (2-Level)/1(ref), Scope/1
  Rate Transition2/1 -> Switch1/3
  Rate Transition1/1 -> Switch1/1

== system sschdlexSolarInverterSingleNetworkModel/Simple Time Delay Sensor ==
  u : Inport
  1/Tau : Gain  Gain=1/Tau
  Discrete-Time Integrator : DiscreteIntegrator  SampleTime=Ts  ICPrevOutput=DiscIntNeverNeededParam  ICPrevScaledInput=DiscIntNeverNeededParam
  Sum : Sum  Inputs=|+-
  y : Outport  VectorParamsAs1DForOutWhenUnconnected=off
  wires:
  1/Tau/1 -> Discrete-Time Integrator/1
  Sum/1 -> 1/Tau/1
  u/1 -> Sum/1
  Discrete-Time Integrator/1 -> y/1, Sum/2

== system sschdlexSolarInverterSingleNetworkModel/Simple Time Delay Sensor  ==
  u : Inport
  1/Tau : Gain  Gain=1/Tau
  Discrete-Time Integrator : DiscreteIntegrator  SampleTime=Ts  ICPrevOutput=DiscIntNeverNeededParam  ICPrevScaledInput=DiscIntNeverNeededParam
  Sum : Sum  Inputs=|+-
  y : Outport  VectorParamsAs1DForOutWhenUnconnected=off
  wires:
  Discrete-Time Integrator/1 -> Sum/2, y/1
  u/1 -> Sum/1
  Sum/1 -> 1/Tau/1
  1/Tau/1 -> Discrete-Time Integrator/1

== system sschdlexSolarInverterSingleNetworkModel/Simple Time Delay Sensor 1 ==
  u : Inport
  1/Tau : Gain  Gain=1/Tau
  Discrete-Time Integrator : DiscreteIntegrator  SampleTime=Ts  ICPrevOutput=DiscIntNeverNeededParam  ICPrevScaledInput=DiscIntNeverNeededParam
  Sum : Sum  Inputs=|+-
  y : Outport  VectorParamsAs1DForOutWhenUnconnected=off
  wires:
  1/Tau/1 -> Discrete-Time Integrator/1
  Sum/1 -> 1/Tau/1
  u/1 -> Sum/1
  Discrete-Time Integrator/1 -> y/1, Sum/2

== system sschdlexSolarInverterSingleNetworkModel/Simple Time Delay Sensor 2 ==
  u : Inport
  1/Tau : Gain  Gain=1/Tau
  Discrete-Time Integrator : DiscreteIntegrator  SampleTime=Ts  ICPrevOutput=DiscIntNeverNeededParam  ICPrevScaledInput=DiscIntNeverNeededParam
  Sum : Sum  Inputs=|+-
  y : Outport  VectorParamsAs1DForOutWhenUnconnected=off
  wires:
  Discrete-Time Integrator/1 -> Sum/2, y/1
  u/1 -> Sum/1
  Sum/1 -> 1/Tau/1
  1/Tau/1 -> Discrete-Time Integrator/1

== system sschdlexSolarInverterSingleNetworkModel/Vfilter ==
  u : Inport
  1/T6 : Gain  Gain=1/Tf
  Discrete-Time Integrator : DiscreteIntegrator  SampleTime=Tc  ICPrevOutput=DiscIntNeverNeededParam  ICPrevScaledInput=DiscIntNeverNeededParam
  Sum1 : Sum  Inputs=|+-
  y : Outport  VectorParamsAs1DForOutWhenUnconnected=off
  wires:
  1/T6/1 -> Discrete-Time Integrator/1
  u/1 -> Sum1/1
  Discrete-Time Integrator/1 -> y/1, Sum1/2
  Sum1/1 -> 1/T6/1

== system sschdlexSolarInverterSingleNetworkModel/Inverter Controls/PWM Generator (2-Level) ==
  ref : Inport  SampleTime=Ts
  Carrier counter : Subsystem  LoadFcn=ee_sli_rtmsupport( 'loadfcn', gcbh );  mask(Counter){CarrCount=Up-Down, Range=Range, Tper=Tper, Tdelay=Td, Ts=Ts}
      mask prompts: CarrCount "physmod:ee:library:comments:control:eeGeneralControl:CounterType_MP"; Range "physmod:ee:library:comments:control:eeGeneralControl:OutputRange_MP"; Tper "physmod:ee:library:comments:control:eeGeneralControl:TimerPeriods_MP"; Tdelay "physmod:ee:library:comments:control:eeGeneralControl:PhaseDelays_MP"; Ts "physmod:ee:library:comments:control:eeGeneralControl:SampleTime_MP"
      mask help: physmod:ee:library:comments:control:eeGeneralControl:Counter_MD
      mask init:
      | timeDomain = ee.mask.getTimeDomain(Ts);
      settings: CopyFcn=ee_sli_rtmsupport( 'copyfcn', gcbh );  DeleteFcn=ee_sli_rtmsupport( 'deletefcn', gcbh );  ModelCloseFcn=ee_sli_rtmsupport( 'modelclosefcn', gcbh );  PostSaveFcn=ee_sli_rtmsupport( 'postsavefcn', gcbh );  PreCopyFcn=ee_sli_rtmsupport( 'precopyfcn', gcbh );  OpenFcn=ee_sli_rtmsupport( 'openfcn', gcbh );  CloseFcn=ee_sli_rtmsupport( 'closefcn', gcbh );  PreDeleteFcn=ee_sli_rtmsupport( 'predeletefcn', gcbh );
      mask Help: web(nesl_help(gcbh))
      mask TypeOptions CarrCount: physmod:ee:library:comments:control:eeGeneralControl:Up_PV | physmod:ee:library:comments:control:eeGeneralControl:Down_PV | physmod:ee:library:comments:control:eeGeneralControl:Up0x2DDown_PV
      mask TypeOptions Ts:
      | Integrator with
      | Wrapped State
      | (Discrete or Continuous)/Ts | Integrator with
      | Wrapped State
      | (Discrete or Continuous)1/Ts
      mask DialogControl ParameterGroupVar Prompt: physmod:ee:library:comments:control:eeGeneralControl:tab_Parameters
      mask DialogControl CarrCount Prompt: Counter type
      mask DialogControl Range Prompt: Output range
      mask DialogControl Tper Prompt: Timer period (s)
      mask DialogControl Tdelay Prompt: Phase delay (s)
      mask DialogControl Ts Prompt: Sample time
  Data Type Conversion2 : DataTypeConversion  SaturateOnIntegerOverflow=off  RndMeth=Floor
  Gain : Gain  Gain=-1
  Logical Operator : Logic  Operator=NOT  AllPortsSameDT=off  OutDataTypeStr=boolean
  Logical Operator1 : Logic  Operator=NOT  AllPortsSameDT=off  OutDataTypeStr=boolean
  Mux : Mux
  Relational Operator : RelationalOperator  OutDataTypeStr=boolean  RndMeth=Simplest  InputSameDT=off
  Relational Operator1 : RelationalOperator  OutDataTypeStr=boolean  RndMeth=Simplest  InputSameDT=off
  Selector : Selector  InputPortWidth=4  IndexOptions=Index vector (dialog)  Indices=PwmOutSelect  OutputSizes=1
  PWM : Outport  VectorParamsAs1DForOutWhenUnconnected=off
  wires:
  Relational Operator1/1 -> Mux/3, Logical Operator1/1
  Data Type Conversion2/1 -> PWM/1
  Relational Operator/1 -> Mux/1, Logical Operator/1
  Gain/1 -> Relational Operator1/1
  Logical Operator1/1 -> Mux/4
  Logical Operator/1 -> Mux/2
  Mux/1 -> Selector/1
  Carrier counter/1(T) -> Relational Operator1/2, Relational Operator/2
  ref/1 -> Gain/1, Relational Operator/1
  Selector/1 -> Data Type Conversion2/1

== system sschdlexSolarInverterSingleNetworkModel/MPPT and Boost Controllers/Digital Pulse ==
  Freq : Inport
  Compare To Constant : simulink/Logic and Bit Operations/Compare To Constant  relop=>=  const=Duty  OutDataTypeStr=boolean
  Constant1 : Constant
  Discrete-Time Integrator : DiscreteIntegrator  ExternalReset=rising  SampleTime=Ts  ShowStatePort=on  ICPrevOutput=DiscIntNeverNeededParam  ICPrevScaledInput=DiscIntNeverNeededParam
  Relational Operator1 : RelationalOperator  Operator=>  OutDataTypeStr=boolean  InputSameDT=off
  Pulse : Outport  VectorParamsAs1DForOutWhenUnconnected=off
  wires:
  Relational Operator1/1 -> Discrete-Time Integrator/2
  Constant1/1 -> Relational Operator1/2
  Compare To Constant/1 -> Pulse/1
  Discrete-Time Integrator/State -> Relational Operator1/1
  Discrete-Time Integrator/1 -> Compare To Constant/1
  Freq/1 -> Discrete-Time Integrator/1
